simulink model "lab2simulink"  (R2024b)
settings: Solver=VariableStepAuto  StartTime=0.0  StopTime=20  MaxStep=.001  RelTol=1e-6
undefined symbols (not defined in the file or in its folder): dspblkCoreblockFVToolHelper, gcbh
settings Model: Creator=kushls2  LastModifiedBy=ttkim2

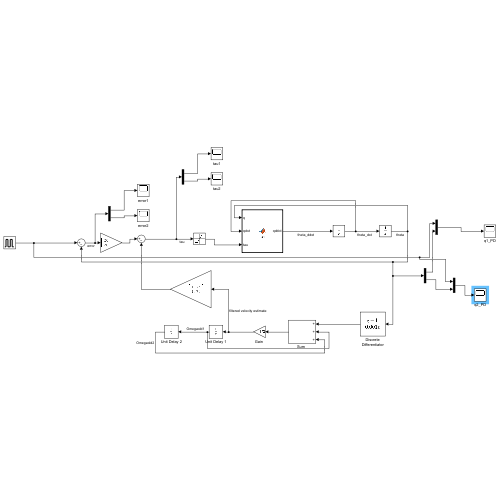
[thumbnail: Simulink's stored preview of the top-level diagram]
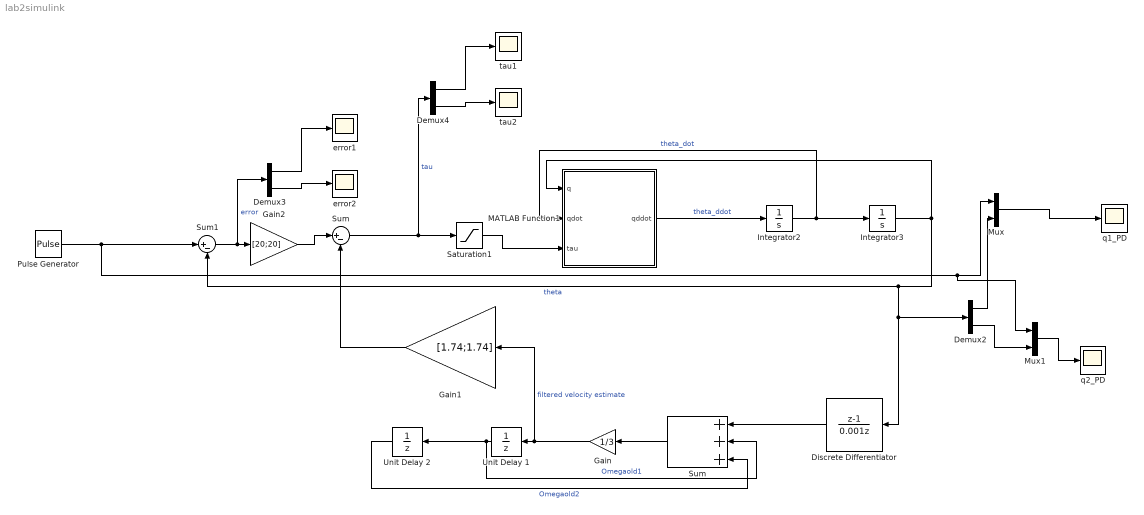
== system lab2simulink ==
  Demux2 : Demux  Outputs=2
  Demux3 : Demux  Outputs=2
  Demux4 : Demux  Outputs=2
  Discrete Differentiator : DiscreteTransferFcn  LoadFcn=dspblkCoreblockFVToolHelper(gcbh,'load');  Numerator=[1 -1]  Denominator=[0.001 0]
      settings: CopyFcn=dspblkCoreblockFVToolHelper(gcbh,'copy');  DeleteFcn=dspblkCoreblockFVToolHelper(gcbh,'close');  ModelCloseFcn=dspblkCoreblockFVToolHelper(gcbh,'close');  PreSaveFcn=dspblkCoreblockFVToolHelper(gcbh,'presave');  PostSaveFcn=dspblkCoreblockFVToolHelper(gcbh,'postsave');  CloseFcn=dspblkCoreblockFVToolHelper(gcbh,'close');
  "Gain " : Gain  Gain=1/3
  Gain1 : Gain  Gain=[1.74;1.74]
  Gain2 : Gain  Gain=[20;20]
  Integrator2 : Integrator  InitialCondition=[0;0]
  Integrator3 : Integrator  InitialCondition=[0;0]
  MATLAB Function1 : MATLAB Function  TreatAsAtomicUnit=on
  Mux : Mux  Inputs=2
  Mux1 : Mux  Inputs=2
  Pulse Generator : DiscretePulseGenerator  PulseType=Time based  Amplitude=0.5  Period=8  PulseWidth=50
  Saturation1 : Saturate  UpperLimit=5  LowerLimit=-5
  Sum : Sum  Inputs=|+-
  "Sum  " : Sum  Inputs=+++
  Sum1 : Sum  Inputs=|+-
  Unit Delay 1 : UnitDelay  SampleTime=0.001  HasFrameUpgradeWarning=on
  Unit Delay 2 : UnitDelay  SampleTime=0.001  HasFrameUpgradeWarning=on
  error1 : Scope
  error2 : Scope
  q1_PD : Scope
  q2_PD : Scope
  tau1 : Scope
  tau2 : Scope
  wires:
  Sum/1 -> Demux4/1, Saturation1/1  "tau"
  Integrator3/1 -> Demux2/1, Discrete Differentiator/1, Sum1/2, MATLAB Function1/1(q)  "theta"
  Integrator2/1 -> MATLAB Function1/2(qdot), Integrator3/1  "theta_dot"
  Discrete Differentiator/1 -> "Sum  "/1
  "Sum  "/1 -> "Gain "/1
  "Gain "/1 -> Gain1/1, Unit Delay 1/1  "filtered velocity estimate"
  Unit Delay 1/1 -> "Sum  "/2, Unit Delay 2/1  "Omegaold1"
  Unit Delay 2/1 -> "Sum  "/3  "Omegaold2"
  Gain1/1 -> Sum/2
  Gain2/1 -> Sum/1
  Sum1/1 -> Demux3/1, Gain2/1  "error"
  Pulse Generator/1 -> Mux1/1, Mux/1, Sum1/1
  Demux3/1 -> error1/1
  Demux3/2 -> error2/1
  Demux4/1 -> tau1/1
  Demux4/2 -> tau2/1
  Saturation1/1 -> MATLAB Function1/3(tau)
  MATLAB Function1/1(qddot) -> Integrator2/1  "theta_ddot"
  Mux/1 -> q1_PD/1
  Demux2/1 -> Mux/2
  Demux2/2 -> Mux1/2
  Mux1/1 -> q2_PD/1

== matlab function lab2simulink/MATLAB Function1 ==
  data: q input; qddot output; qdot input; tau input
function qddot = fcn(q, qdot, tau)
p1 = 0.03;
p2 = 0.0128;
p3 = 0.0076;
p4 = 0.0753;
p5 = 0.0298;
g  = 9.81;


theta2  = q(1);
dtheta2 = qdot(1);
theta3  = q(2);
dtheta3 = qdot(2);

d = theta3 - theta2;

D = [ p1,           -p3*sin(d);
     -p3*sin(d),     p2      ];

C = [ 0,                 -p3*cos(d)*dtheta3;
      p3*cos(d)*dtheta2,  0               ];

G = [ -p4*g*sin(theta2);
      -p5*g*cos(theta3) ];


qddot = (inv(D)*tau - inv(D)*C*qdot - inv(D)*G);
